simulink model "MixerSimple_LogIMU_RawDatas_30f4012"  (Simulink 7.2)
settings: Solver=FixedStepDiscrete  StartTime=0.0  StopTime=10.0  FixedStep=0.001  RelTol=1e-3
undefined symbols (not defined in the file or in its folder): IC1max, PWM
libraries: dsPICdrivers x42, simulink x31
CloseFcn:
  | rtwprivate ssgencode ModelCloseRequest Autopilote_30f4012
settings Model: Creator=Lubin  LastModifiedBy=Administrateur
settings OptimizationCC: InlineParams=on  InitFltsAndDblsToZero=on  OptimizeModelRefInitCode=on  LifeSpan=1
settings DebuggingCC: SaveWithParameterizedLinksMsg=none
settings HardwareCC: ProdBitPerInt=16  ProdEndianess=LittleEndian  ProdWordSize=16  ProdHWDeviceType=16-bit Generic
settings RTWCC: SystemTargetFile=dspic.tlc  TemplateMakefile=dspic_pic30_gcc.tmf  PostCodeGenCommand=dsPIC_Compile()  Description=Embedded Target for Microchip dsPIC (real-time)  GenerateReport=on  ProcessScript=dspic_make_rtw_hook  IncludeHyperlinkInReport=on  LaunchReport=on  GenerateTraceInfo=on  GenerateTraceReport=on  GenerateTraceReportSl=on  GenerateTraceReportSf=on  GenerateTraceReportEml=on
settings CodeAppCC: IgnoreCustomStorageClasses=off
settings STFCustomTargetCC: ModelReferenceCompliant=off  IncludeMdlTerminateFcn=off  CombineOutputUpdateFcns=on  SuppressErrorStatus=on  ERTCustomFileBanners=on  SupportContinuousTime=off  SupportNonInlinedSFcns=off  CPPClassGenCompliant=on  SystemTargetFile=dspic.tlc
settings ERTTargetCC: MultiwordLength=2048  ModelReferenceCompliant=off  CompOptLevelCompliant=off  IncludeMdlTerminateFcn=off  SuppressErrorStatus=on  ERTFirstTimeCompliant=off  ModelStepFunctionPrototypeControlCompliant=off  InlinedParameterPlacement=NonHierarchical  ERTSrcFileBannerTemplate=dsPIC_code_template.cgt  ERTHdrFileBannerTemplate=dsPIC_code_template.cgt  ERTDataSrcFileTemplate=dsPIC_code_template.cgt  ERTDataHdrFileTemplate=dsPIC_code_template.cgt  ERTCustomFileTemplate=dsPIC_main.tlc
settings CustomProperty: DataType=string  Value=C:\PROGRA~1\MATLAB\R2008a\bin\win32\gmake

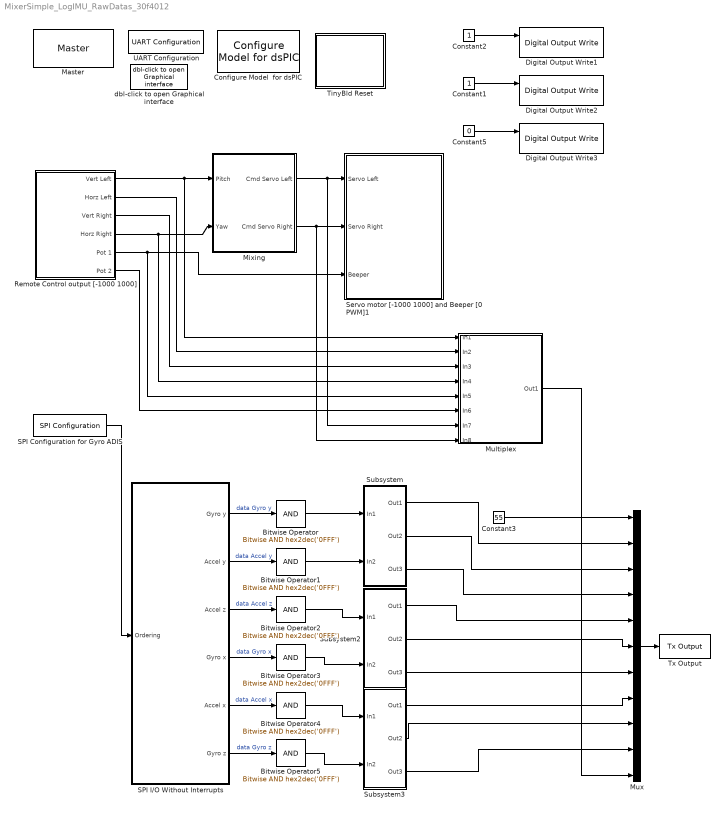
== system MixerSimple_LogIMU_RawDatas_30f4012 ==
  Bitwise Operator{,1..5} (6 alike) : simulink/Logic and Bit Operations/Bitwise Operator  logicop=AND  UseBitMask=on  BitMask=hex2dec('0FFF')  BitMaskRealWorld=Stored Integer
  Configure Model  for dsPIC : dsPICdrivers/Simulink Configuration/Configure Model  for dsPIC
  Constant1 : Constant  OutDataTypeMode=boolean  OutDataType=sfix(16)  OutScaling=2^0  OutDataTypeStr=boolean
  Constant2 : Constant  OutDataTypeMode=boolean  OutDataType=sfix(16)  OutScaling=2^0  OutDataTypeStr=boolean
  Constant3 : Constant  Value=55  OutDataTypeMode=uint8  OutDataType=sfix(16)  OutScaling=2^0  OutDataTypeStr=uint8  SampleTime=-1
  Constant5 : Constant  Value=0  OutDataTypeMode=boolean  OutDataType=sfix(16)  OutScaling=2^0  OutDataTypeStr=boolean
  Digital Output Write1 : dsPICdrivers/Digital I//O/Digital Output Write  Tag=dsPIC_Digital_Output  Priority=5  PORT=E  Pin=5  Simultaneous=off  OrderingInOutPopup=Input & Output
  Digital Output Write2 : dsPICdrivers/Digital I//O/Digital Output Write  Tag=dsPIC_Digital_Output  Priority=5  PORT=E  Pin=3  Simultaneous=off  OrderingInOutPopup=Input & Output
  Digital Output Write3 : dsPICdrivers/Digital I//O/Digital Output Write  Tag=dsPIC_Digital_Output  Priority=5  PORT=E  Pin=1  Simultaneous=off  OrderingInOutPopup=Input
  Master : dsPICdrivers/Master  Tag=dsPIC_MASTER  Priority=1  TimeStepType=Timer1  picType=30f4012  fcy=20e6  Quartz_33f=5e6  PLLActive_33f=off  fcyDesired_33f=0  tmr1="[1  19999  0]"  tmr1Info="Time Step : 0.001  ;   Error : 0%  PR1=19999"  tmr2345="[1  0  0  0]"  tmr2345cfg=[-1 -1 -1 -1]  IOautoConf=on  typePort="[ 0   0   0   0   0   0   0   0   0   0   0   0   0   0   0   0  10   0  13  13   6   6   0   0   0   0   0   0   0   0   0   0   0   0   0   0   0   0   0   0   0   0   0   0   0   5   4   0   6   6   0   0   0   0   0   0   0   0   0   0   0   0   0   0  11  10  11  10  11  10   0   0  17   0   0   0   0   0   0   0   0   0  14  15   0   0   0   0   0   0   0   0   0   0   0   0   0   0   0   0   0   0   0   0   0   0   0   0   0   0   0   0 ]"  TRIS="[ 65535  65534  65535  65535  65493  65535  65535 ]"  ADPCFG=61  MasterBusyPort=None  MasterOverloadPort=None  FOSC=XT_PLL8  ClockSwitchMonitor=Both disabled  TempProtection_33f=TEMP_ON  FPBOR=PBOR_OFF  PWRT=PWRT_4  MCLR=MCLR_DIS  PowerSave=off  OverrideFcy=off  NewFcy=1e6
  Mixing : Subsystem
  Multiplex : Subsystem
  Mux : Mux  Inputs=11
  Remote Control output [-1000 1000] : Subsystem
  SPI Configuration for Gyro ADIS : dsPICdrivers/SPI PORT/SPI Configuration  Tag=dsPIC_config_SPI  Priority=2  ConfigurationTime=At block execution (reconfigure on the fly)  OrderingInOutPopup=Output  SampleTime=-1  Frame_Enable=0  Frame_Sync=0  SPI=1  MODE=MASTER  USER_SCALER=2  StartEnable=Enable  SDO_EN=on  DATA_LENGTH=16 bits  SS_EN=off  SMP=Middle of bit  CKP=high  CKE=Idle to Active  Status="OK - Mode 1  -    Fsck= 10000000Hz"
  SPI I/O Without Interrupts : Subsystem
  Servo motor [-1000 1000] and Beeper [0 PWM]1 : Subsystem
  Subsystem : Subsystem
  Subsystem2 : Subsystem
  Subsystem3 : Subsystem
  TinyBld Reset : Subsystem  AncestorBlock=dsPICdrivers/OTHERS/TinyBld Reset
      mask Display: fprintf('TinyBld\nReset')
  Tx Output : dsPICdrivers/Serial PORT/Tx Output  Tag=dsPIC_TX  Priority=5  UART=1  OrderingInOutPopup=None
  UART Configuration : dsPICdrivers/Serial PORT/UART Configuration  Tag=dsPIC_config_UART  Priority=2  UART=1  proposed_BAUD=115200  ALT_TX_RX=on  InterruptTxWhen=When Transmit Buffer is empty  TXInterruptPri=1  TxBufferSize=32  TXEN=on  InterruptRxWhen=When Receive Buffer is full (contain 4 characters)  RXInterruptPri=1  RxBufferSize=32  BAUD=115200  UxBRG=10  Info="UxBRG = 10   ||  Real Baud : 113636   ||  % error : -1.3573  ||  max 11.3636 Bytes / Step"  RealBaud=0
  dbl-click to open Graphical interface : dsPICdrivers/Serial PORT/dbl-click to open Graphical interface  SystemSampleTime=-1  Nothing=0
  wires:
  Constant2/1 -> Digital Output Write1/1
  Constant1/1 -> Digital Output Write2/1
  Constant5/1 -> Digital Output Write3/1
  SPI Configuration for Gyro ADIS/1 -> SPI I/O Without Interrupts/1(Ordering)
  SPI I/O Without Interrupts/1(Gyro y) -> Bitwise Operator/1  "data Gyro y"
  SPI I/O Without Interrupts/2(Accel y) -> Bitwise Operator1/1  "data Accel y"
  SPI I/O Without Interrupts/3(Accel z) -> Bitwise Operator2/1  "data Accel z"
  SPI I/O Without Interrupts/4(Gyro x) -> Bitwise Operator3/1  "data Gyro x"
  SPI I/O Without Interrupts/5(Accel x) -> Bitwise Operator4/1  "data Accel x"
  SPI I/O Without Interrupts/6(Gyro z) -> Bitwise Operator5/1  "data Gyro z"
  Bitwise Operator/1 -> Subsystem/1(In1)
  Bitwise Operator1/1 -> Subsystem/2(In2)
  Bitwise Operator2/1 -> Subsystem2/1(In1)
  Bitwise Operator3/1 -> Subsystem2/2(In2)
  Bitwise Operator4/1 -> Subsystem3/1(In1)
  Bitwise Operator5/1 -> Subsystem3/2(In2)
  Mux/1 -> Tx Output/1
  Constant3/1 -> Mux/1
  Subsystem/1(Out1) -> Mux/2
  Subsystem/2(Out2) -> Mux/3
  Subsystem/3(Out3) -> Mux/4
  Subsystem2/1(Out1) -> Mux/5
  Subsystem2/2(Out2) -> Mux/6
  Subsystem2/3(Out3) -> Mux/7
  Subsystem3/1(Out1) -> Mux/8
  Subsystem3/2(Out2) -> Mux/9
  Subsystem3/3(Out3) -> Mux/10
  Mixing/1(Cmd Servo Left) -> Servo motor [-1000 1000] and Beeper [0 PWM]1/1(Servo Left), Multiplex/7(In7)
  Remote Control output [-1000 1000]/1(Vert Left) -> Mixing/1(Pitch), Multiplex/1(In1)
  Remote Control output [-1000 1000]/4(Horz Right) -> Mixing/2(Yaw), Multiplex/4(In4)
  Mixing/2(Cmd Servo Right) -> Servo motor [-1000 1000] and Beeper [0 PWM]1/2(Servo Right), Multiplex/8(In8)
  Remote Control output [-1000 1000]/5(Pot 1) -> Servo motor [-1000 1000] and Beeper [0 PWM]1/3(Beeper), Multiplex/5(In5)
  Remote Control output [-1000 1000]/2(Horz Left) -> Multiplex/2(In2)
  Remote Control output [-1000 1000]/3(Vert Right) -> Multiplex/3(In3)
  Remote Control output [-1000 1000]/6(Pot 2) -> Multiplex/6(In6)
  Multiplex/1(Out1) -> Mux/11

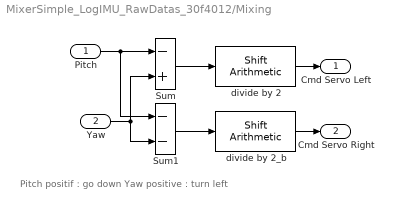
== system MixerSimple_LogIMU_RawDatas_30f4012/Mixing ==
  note: Pitch positif : go down
      | Yaw positive : turn left
  Pitch : Inport
  Yaw : Inport  Port=2
  Sum : Sum  Inputs=-+  AccumDataTypeStr=int16  OutDataTypeMode=int16  OutDataType=sfix(16)  OutScaling=2^0  OutDataTypeStr=int16  SaturateOnIntegerOverflow=on  InputSameDT=on
  Sum1 : Sum  Inputs=--  AccumDataTypeStr=int16  OutDataTypeMode=int16  OutDataType=sfix(16)  OutScaling=2^0  OutDataTypeStr=int16  SaturateOnIntegerOverflow=on  InputSameDT=on
  divide by 2 : simulink/Logic and Bit Operations/Shift Arithmetic  SystemSampleTime=-1  nBitShiftRight=1  nBinPtShiftRight=0
  divide by 2_b : simulink/Logic and Bit Operations/Shift Arithmetic  SystemSampleTime=-1  nBitShiftRight=1  nBinPtShiftRight=0
  Cmd Servo Left : Outport
  Cmd Servo Right : Outport  Port=2
  wires:
  divide by 2_b/1 -> Cmd Servo Right/1
  divide by 2/1 -> Cmd Servo Left/1
  Yaw/1 -> Sum/2, Sum1/2
  Sum1/1 -> divide by 2_b/1
  Sum/1 -> divide by 2/1
  Pitch/1 -> Sum/1, Sum1/1

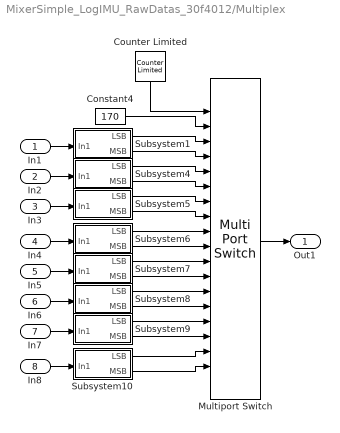
== system MixerSimple_LogIMU_RawDatas_30f4012/Multiplex ==
  In1 : Inport
  In2 : Inport  Port=2
  In3 : Inport  Port=3
  In4 : Inport  Port=4
  In5 : Inport  Port=5
  In6 : Inport  Port=6
  In7 : Inport  Port=7
  In8 : Inport  Port=8
  Constant4 : Constant  Value=170  OutDataTypeMode=uint8  OutDataType=sfix(16)  OutScaling=2^0  OutDataTypeStr=uint8  SampleTime=-1
  Counter Limited : simulink/Sources/Counter Limited  Orientation=down  SystemSampleTime=-1  uplimit=16  tsamp=-1
  Multiport Switch : MultiPortSwitch  Inputs=17  OutDataType=sfix(16)  OutScaling=2^0
  Subsystem1 : Subsystem
  Subsystem10 : Subsystem
  Subsystem4 : Subsystem
  Subsystem5 : Subsystem
  Subsystem6 : Subsystem
  Subsystem7 : Subsystem
  Subsystem8 : Subsystem
  Subsystem9 : Subsystem
  Out1 : Outport
  wires:
  Counter Limited/1 -> Multiport Switch/1
  Constant4/1 -> Multiport Switch/2
  Subsystem1/1(LSB) -> Multiport Switch/3
  Subsystem1/2(MSB) -> Multiport Switch/4
  Subsystem4/1(LSB) -> Multiport Switch/5
  Subsystem4/2(MSB) -> Multiport Switch/6
  Subsystem5/1(LSB) -> Multiport Switch/7
  Subsystem5/2(MSB) -> Multiport Switch/8
  Subsystem6/1(LSB) -> Multiport Switch/9
  Subsystem6/2(MSB) -> Multiport Switch/10
  Subsystem7/1(LSB) -> Multiport Switch/11
  Subsystem7/2(MSB) -> Multiport Switch/12
  Subsystem8/1(LSB) -> Multiport Switch/13
  Subsystem8/2(MSB) -> Multiport Switch/14
  Subsystem9/1(LSB) -> Multiport Switch/15
  Subsystem9/2(MSB) -> Multiport Switch/16
  Subsystem10/1(LSB) -> Multiport Switch/17
  Subsystem10/2(MSB) -> Multiport Switch/18
  In1/1 -> Subsystem1/1(In1)
  In2/1 -> Subsystem4/1(In1)
  In3/1 -> Subsystem5/1(In1)
  In4/1 -> Subsystem6/1(In1)
  Multiport Switch/1 -> Out1/1
  In5/1 -> Subsystem7/1(In1)
  In6/1 -> Subsystem8/1(In1)
  In7/1 -> Subsystem9/1(In1)
  In8/1 -> Subsystem10/1(In1)

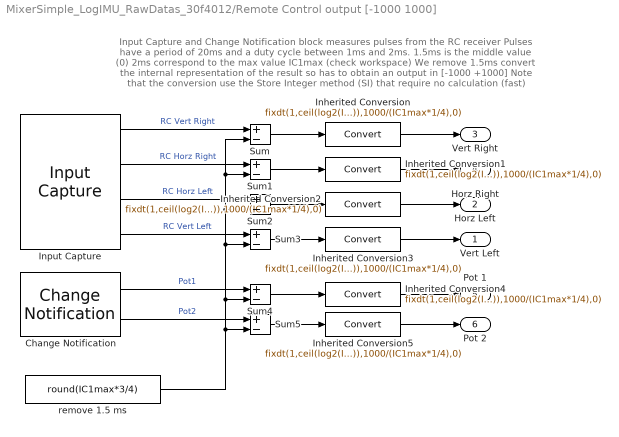
== system MixerSimple_LogIMU_RawDatas_30f4012/Remote Control output [-1000 1000] ==
  note: Input Capture and Change Notification block measures pulses from the RC receiver
      | Pulses have a period of 20ms and a duty cycle between 1ms and 2ms. 1.5ms is the middle value (0)
      | 2ms correspond to the max value IC1max (check workspace)
      | We remove 1.5ms convert the internal representation of the result so has to obtain an output in [-1000 +1000]
      | Note that the conversion use the Store Integer method (SI) that require no calculation (fast)
  Change Notification : dsPICdrivers/Peripheral I//O/Change Notification  Tag=dsPIC_PWM_CN  Priority=5  IntPriority=7  Channel="[4 5  ]"  Pin="[2  3]"  NumPort="[1  1]"  Channel_UP_Down_Periode="[1  1]"  MaxChannel="[0.002       0.002]"  SafeMarge="[10  10]"  MaxName=' CN4max , CN5max '  Precision="[15.2877      15.2877]"  Timer="[2  2]"  ChangeDetected="[0  0]"  PullUp="[0  0]"  SampleTime=.001  Status=OK
  Inherited Conversion{,1..5} (6 alike) : DataTypeConversion  OutDataTypeMode=Specify via dialog  OutDataType=fixdt(1,ceil(log2(IC1max*1/4)),1000/(IC1max*1/4),0)  OutDataTypeStr=fixdt(1,ceil(log2(IC1max*1/4)),1000/(IC1max*1/4),0)  ConvertRealWorld=Stored Integer (SI)  LockScale=on
  Input Capture : dsPICdrivers/Peripheral I//O/Input Capture  Tag=dsPIC_PWM_IC  Priority=5  IntPriority=7  Channel=[1 2 7 8 ]  Channel_UP_Down_Periode="[1  1  1  1]"  MaxChannel="[0.002       0.002       0.002       0.002]"  SafeMarge="[10  10  10  10]"  MaxName=' IC1max , IC2max , IC7max , IC8max '  Precision="[15.2877      15.2877      15.2877      15.2877]"  Timer="[2  2  2  2]"  ChangeDetected="[0  0  0  0]"  ChangeDetectedPortRef=0  SampleTime=.001  Status=OK
  Sum{,1..5} (6 alike) : Sum  Inputs=+-  AccumDataTypeStr=uint16  OutDataTypeMode=int16  OutDataType=sfix(16)  OutScaling=2^0  OutDataTypeStr=int16  InputSameDT=on
  remove 1.5 ms : Constant  Value=round(IC1max*3/4)  OutDataTypeMode=uint16  OutDataType=sfix(16)  OutScaling=2^0  OutDataTypeStr=uint16
  Vert Left : Outport
  Horz Left : Outport  Port=2
  Vert Right : Outport  Port=3
  Horz Right : Outport  Port=4
  Pot 1 : Outport  Port=5
  Pot 2 : Outport  Port=6
  wires:
  Input Capture/1 -> Sum/1  "RC Vert Right"
  Input Capture/2 -> Sum1/1  "RC Horz Right"
  Input Capture/3 -> Sum2/1  "RC Horz Left"
  Input Capture/4 -> Sum3/1  "RC Vert Left"
  Change Notification/1 -> Sum4/1  "Pot1"
  Change Notification/2 -> Sum5/1  "Pot2"
  remove 1.5 ms/1 -> Sum5/2, Sum/2, Sum1/2, Sum2/2, Sum3/2, Sum4/2
  Sum/1 -> Inherited Conversion/1
  Inherited Conversion/1 -> Vert Right/1
  Sum3/1 -> Inherited Conversion3/1
  Sum1/1 -> Inherited Conversion1/1
  Sum2/1 -> Inherited Conversion2/1
  Inherited Conversion1/1 -> Horz Right/1
  Inherited Conversion2/1 -> Horz Left/1
  Inherited Conversion3/1 -> Vert Left/1
  Sum4/1 -> Inherited Conversion4/1
  Sum5/1 -> Inherited Conversion5/1
  Inherited Conversion4/1 -> Pot 1/1
  Inherited Conversion5/1 -> Pot 2/1

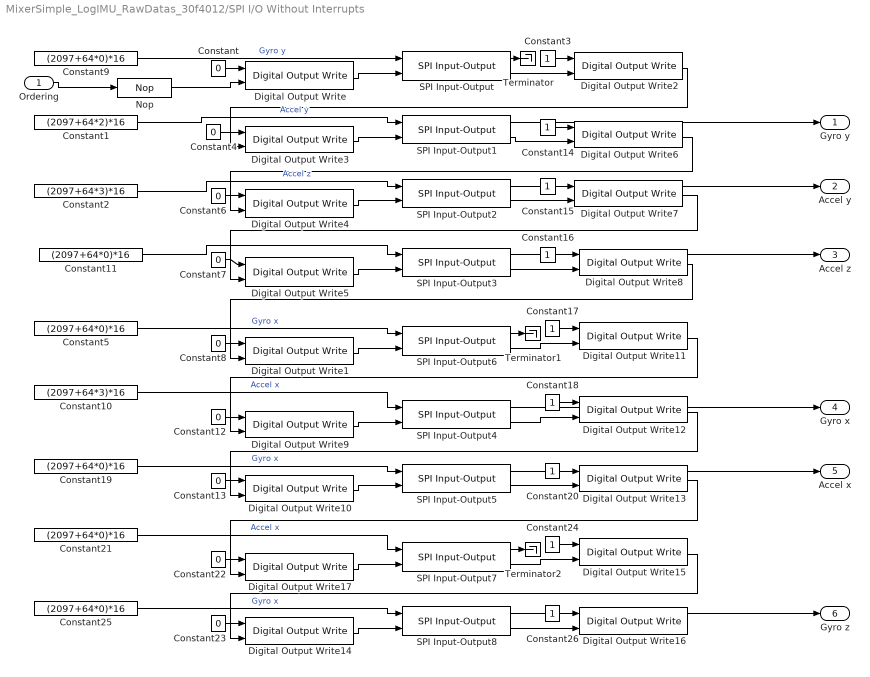
== system MixerSimple_LogIMU_RawDatas_30f4012/SPI I/O Without Interrupts ==
  Ordering : Inport  OutDataType=sfix(16)  OutScaling=2^0
  Constant{,4,6..8,12..13,22..23} (9 alike) : Constant  Value=0  OutDataTypeMode=boolean  OutDataType=sfix(16)  OutScaling=2^0  OutDataTypeStr=boolean
  Constant1 : Constant  Value=(2097+64*2)*16  VectorParams1D=off  OutDataTypeMode=uint16  OutDataType=sfix(16)  OutScaling=2^0  OutDataTypeStr=uint16  SampleTime=-1
  Constant10 : Constant  Value=(2097+64*3)*16  VectorParams1D=off  OutDataTypeMode=uint16  OutDataType=sfix(16)  OutScaling=2^0  OutDataTypeStr=uint16  SampleTime=-1
  Constant{5,9,11,19,21,25} (6 alike) : Constant  Value=(2097+64*0)*16  VectorParams1D=off  OutDataTypeMode=uint16  OutDataType=sfix(16)  OutScaling=2^0  OutDataTypeStr=uint16  SampleTime=-1
  Constant{3,14..18,20,24,26} (9 alike) : Constant  OutDataTypeMode=boolean  OutDataType=sfix(16)  OutScaling=2^0  OutDataTypeStr=boolean
  Constant2 : Constant  Value=(2097+64*3)*16  VectorParams1D=off  OutDataTypeMode=uint16  OutDataType=sfix(16)  OutScaling=2^0  OutDataTypeStr=uint16  SampleTime=-1
  Digital Output Write{,2..8} (8 alike) : dsPICdrivers/Digital I//O/Digital Output Write  Tag=dsPIC_Digital_Output  Priority=5  PORT=E  Pin=5  Simultaneous=off  OrderingInOutPopup=Input & Output
  Digital Output Write{1,9..13} (6 alike) : dsPICdrivers/Digital I//O/Digital Output Write  Tag=dsPIC_Digital_Output  Priority=5  PORT=E  Pin=3  Simultaneous=off  OrderingInOutPopup=Input & Output
  Digital Output Write14 : dsPICdrivers/Digital I//O/Digital Output Write  Tag=dsPIC_Digital_Output  Priority=5  PORT=B  Pin=0  Simultaneous=off  OrderingInOutPopup=Input & Output
  Digital Output Write15 : dsPICdrivers/Digital I//O/Digital Output Write  Tag=dsPIC_Digital_Output  Priority=5  PORT=B  Pin=0  Simultaneous=off  OrderingInOutPopup=Input & Output
  Digital Output Write16 : dsPICdrivers/Digital I//O/Digital Output Write  Tag=dsPIC_Digital_Output  Priority=5  PORT=B  Pin=0  Simultaneous=off  OrderingInOutPopup=Input
  Digital Output Write17 : dsPICdrivers/Digital I//O/Digital Output Write  Tag=dsPIC_Digital_Output  Priority=5  PORT=B  Pin=0  Simultaneous=off  OrderingInOutPopup=Input & Output
  Nop : dsPICdrivers/OTHERS/Nop  Tag=dsPIC_Reset  NbrNop=30
  SPI Input-Output{,1..8} (9 alike) : dsPICdrivers/SPI PORT/SPI Input-Output  Tag=dsPIC_SPI  SPI=1  INPUT=on  RESET_INPUT=off  OUTPUT=on  SPECIAL_SPI=Always Enable  DATA_LENGTH=16 bits  WAIT_INPUTDATA=on  OrderingInOutPopup=Input & Output  SampleTime=-1
  Terminator : Terminator
  Terminator1 : Terminator
  Terminator2 : Terminator
  Gyro y : Outport
  Accel y : Outport  Port=2
  Accel z : Outport  Port=3
  Gyro x : Outport  Port=4
  Accel x : Outport  Port=5
  Gyro z : Outport  Port=6
  wires:
  SPI Input-Output6/1 -> Terminator1/1
  SPI Input-Output/1 -> Terminator/1
  SPI Input-Output5/1 -> Accel x/1
  SPI Input-Output4/1 -> Gyro x/1
  SPI Input-Output3/1 -> Accel z/1
  SPI Input-Output2/1 -> Accel y/1
  SPI Input-Output1/1 -> Gyro y/1
  Digital Output Write12/1 -> Digital Output Write10/2
  Digital Output Write11/1 -> Digital Output Write9/2
  SPI Input-Output5/2 -> Digital Output Write13/2
  SPI Input-Output4/2 -> Digital Output Write12/2
  SPI Input-Output6/2 -> Digital Output Write11/2
  Constant20/1 -> Digital Output Write13/1
  Constant18/1 -> Digital Output Write12/1
  Constant17/1 -> Digital Output Write11/1
  Digital Output Write8/1 -> Digital Output Write1/2
  Digital Output Write10/1 -> SPI Input-Output5/2
  Digital Output Write9/1 -> SPI Input-Output4/2
  Digital Output Write1/1 -> SPI Input-Output6/2
  Constant13/1 -> Digital Output Write10/1
  Constant12/1 -> Digital Output Write9/1
  Constant8/1 -> Digital Output Write1/1
  Digital Output Write7/1 -> Digital Output Write5/2
  Digital Output Write6/1 -> Digital Output Write4/2
  SPI Input-Output3/2 -> Digital Output Write8/2
  SPI Input-Output2/2 -> Digital Output Write7/2
  Constant16/1 -> Digital Output Write8/1
  Constant15/1 -> Digital Output Write7/1
  SPI Input-Output1/2 -> Digital Output Write6/2
  Constant14/1 -> Digital Output Write6/1
  Digital Output Write2/1 -> Digital Output Write3/2
  Digital Output Write3/1 -> SPI Input-Output1/2
  Constant4/1 -> Digital Output Write3/1
  Digital Output Write5/1 -> SPI Input-Output3/2
  Constant7/1 -> Digital Output Write5/1
  Digital Output Write4/1 -> SPI Input-Output2/2
  Constant6/1 -> Digital Output Write4/1
  Digital Output Write/1 -> SPI Input-Output/2
  SPI Input-Output/2 -> Digital Output Write2/2
  Constant3/1 -> Digital Output Write2/1
  Constant/1 -> Digital Output Write/1
  Constant9/1 -> SPI Input-Output/1  "Gyro y"
  Constant1/1 -> SPI Input-Output1/1  "Accel y"
  Constant2/1 -> SPI Input-Output2/1  "Accel z"
  Constant11/1 -> SPI Input-Output3/1
  Constant5/1 -> SPI Input-Output6/1  "Gyro x"
  Constant10/1 -> SPI Input-Output4/1  "Accel x"
  Constant19/1 -> SPI Input-Output5/1  "Gyro x"
  Ordering/1 -> Nop/1
  Nop/1 -> Digital Output Write/2
  SPI Input-Output8/1 -> Gyro z/1
  Digital Output Write15/1 -> Digital Output Write14/2
  Digital Output Write13/1 -> Digital Output Write17/2
  SPI Input-Output8/2 -> Digital Output Write16/2
  SPI Input-Output7/2 -> Digital Output Write15/2
  Constant26/1 -> Digital Output Write16/1
  Constant24/1 -> Digital Output Write15/1
  Digital Output Write14/1 -> SPI Input-Output8/2
  Digital Output Write17/1 -> SPI Input-Output7/2
  Constant23/1 -> Digital Output Write14/1
  Constant22/1 -> Digital Output Write17/1
  Constant21/1 -> SPI Input-Output7/1  "Accel x"
  Constant25/1 -> SPI Input-Output8/1  "Gyro x"
  SPI Input-Output7/1 -> Terminator2/1

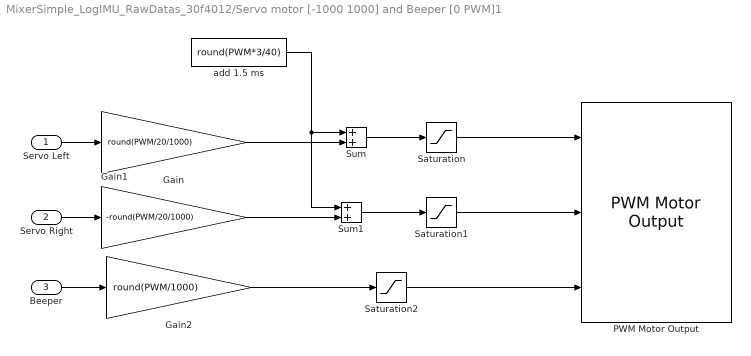
== system MixerSimple_LogIMU_RawDatas_30f4012/Servo motor [-1000 1000] and Beeper [0 PWM]1 ==
  Servo Left : Inport
  Servo Right : Inport  Port=2
  Beeper : Inport  Port=3
  Gain : Gain  Gain=round(PWM/20/1000)  ParameterDataType=sfix(16)  ParameterScaling=2^0  OutDataTypeMode=int16  OutDataType=sfix(16)  OutScaling=2^0  OutDataTypeStr=int16
  Gain1 : Gain  Gain=-round(PWM/20/1000)  ParameterDataType=sfix(16)  ParameterScaling=2^0  OutDataTypeMode=int16  OutDataType=sfix(16)  OutScaling=2^0  OutDataTypeStr=int16
  Gain2 : Gain  Gain=round(PWM/1000)  ParameterDataType=sfix(16)  ParameterScaling=2^0  OutDataTypeMode=uint16  OutDataType=sfix(16)  OutScaling=2^0  OutDataTypeStr=uint16  SaturateOnIntegerOverflow=on
  PWM Motor Output : dsPICdrivers/Peripheral I//O/PWM Motor Output  Tag=dsPIC_PWM_Motor  Priority=5  InputEnableChk=off  InputPeriodeChk=off  Channel=[1 2 3]  TPeriode=.02  PrescalerValue=16  PeriodeInteger=25000  MaxName='PWM'  Centered=off  HChannelON=off  Info="Nbr Bits : 15.6096  ||  PWM = 50000  ||  Prescaler = 16"  Delay=0  IntPriority=5  nbrPwmChannelPIC=3  Status=OK
  Saturation : Saturate  UpperLimit=2*PWM/20  LowerLimit=1*PWM/20  OutDataType=sfix(16)  OutScaling=2^0
  Saturation1 : Saturate  UpperLimit=2*PWM/20  LowerLimit=1*PWM/20  OutDataType=sfix(16)  OutScaling=2^0
  Saturation2 : Saturate  UpperLimit=PWM  LowerLimit=0  OutDataType=sfix(16)  OutScaling=2^0
  Sum : Sum  AccumDataTypeStr=int16  OutDataTypeMode=uint16  OutDataType=sfix(16)  OutScaling=2^0  OutDataTypeStr=uint16
  Sum1 : Sum  AccumDataTypeStr=int16  OutDataTypeMode=uint16  OutDataType=sfix(16)  OutScaling=2^0  OutDataTypeStr=uint16
  add 1.5 ms : Constant  Value=round(PWM*3/40)  OutDataTypeMode=uint16  OutDataType=sfix(16)  OutScaling=2^0  OutDataTypeStr=uint16
  wires:
  Saturation1/1 -> PWM Motor Output/2
  Saturation/1 -> PWM Motor Output/1
  Saturation2/1 -> PWM Motor Output/3
  Gain2/1 -> Saturation2/1
  Beeper/1 -> Gain2/1
  add 1.5 ms/1 -> Sum1/1, Sum/1
  Gain/1 -> Sum/2
  Gain1/1 -> Sum1/2
  Sum1/1 -> Saturation1/1
  Sum/1 -> Saturation/1
  Servo Right/1 -> Gain1/1
  Servo Left/1 -> Gain/1

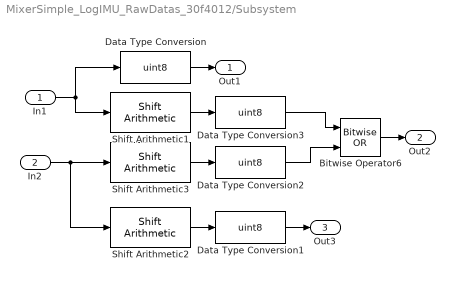
== system MixerSimple_LogIMU_RawDatas_30f4012/Subsystem ==
  In1 : Inport
  In2 : Inport  Port=2
  Bitwise Operator6 : simulink/Logic and Bit Operations/Bitwise Operator  logicop=OR  UseBitMask=off  NumInputPorts=2  BitMask=bin2dec('11011001')  BitMaskRealWorld=Stored Integer
  Data Type Conversion{,1..3} (4 alike) : DataTypeConversion  OutDataTypeMode=uint8  OutDataType=sfix(16)  OutScaling=2^0  OutDataTypeStr=uint8  ConvertRealWorld=Stored Integer (SI)
  Shift Arithmetic1 : simulink/Logic and Bit Operations/Shift Arithmetic  SystemSampleTime=-1  nBitShiftRight=8  nBinPtShiftRight=0
  Shift Arithmetic2 : simulink/Logic and Bit Operations/Shift Arithmetic  SystemSampleTime=-1  nBitShiftRight=4  nBinPtShiftRight=0
  Shift Arithmetic3 : simulink/Logic and Bit Operations/Shift Arithmetic  SystemSampleTime=-1  nBitShiftRight=-4  nBinPtShiftRight=0
  Out1 : Outport
  Out2 : Outport  Port=2
  Out3 : Outport  Port=3
  wires:
  Data Type Conversion3/1 -> Bitwise Operator6/1
  Data Type Conversion1/1 -> Out3/1
  Bitwise Operator6/1 -> Out2/1
  Data Type Conversion/1 -> Out1/1
  Shift Arithmetic1/1 -> Data Type Conversion3/1
  Data Type Conversion2/1 -> Bitwise Operator6/2
  Shift Arithmetic3/1 -> Data Type Conversion2/1
  Shift Arithmetic2/1 -> Data Type Conversion1/1
  In2/1 -> Shift Arithmetic2/1, Shift Arithmetic3/1
  In1/1 -> Data Type Conversion/1, Shift Arithmetic1/1

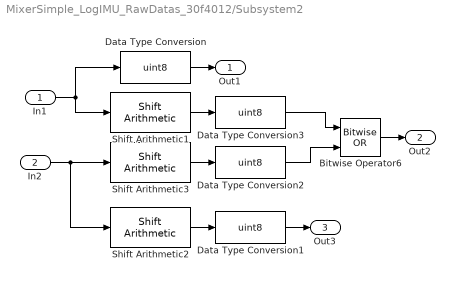
== system MixerSimple_LogIMU_RawDatas_30f4012/Subsystem2 ==
  In1 : Inport
  In2 : Inport  Port=2
  Bitwise Operator6 : simulink/Logic and Bit Operations/Bitwise Operator  logicop=OR  UseBitMask=off  NumInputPorts=2  BitMask=bin2dec('11011001')  BitMaskRealWorld=Stored Integer
  Data Type Conversion{,1..3} (4 alike) : DataTypeConversion  OutDataTypeMode=uint8  OutDataType=sfix(16)  OutScaling=2^0  OutDataTypeStr=uint8  ConvertRealWorld=Stored Integer (SI)
  Shift Arithmetic1 : simulink/Logic and Bit Operations/Shift Arithmetic  SystemSampleTime=-1  nBitShiftRight=8  nBinPtShiftRight=0
  Shift Arithmetic2 : simulink/Logic and Bit Operations/Shift Arithmetic  SystemSampleTime=-1  nBitShiftRight=4  nBinPtShiftRight=0
  Shift Arithmetic3 : simulink/Logic and Bit Operations/Shift Arithmetic  SystemSampleTime=-1  nBitShiftRight=-4  nBinPtShiftRight=0
  Out1 : Outport
  Out2 : Outport  Port=2
  Out3 : Outport  Port=3
  wires:
  In1/1 -> Shift Arithmetic1/1, Data Type Conversion/1
  In2/1 -> Shift Arithmetic3/1, Shift Arithmetic2/1
  Shift Arithmetic2/1 -> Data Type Conversion1/1
  Shift Arithmetic3/1 -> Data Type Conversion2/1
  Data Type Conversion2/1 -> Bitwise Operator6/2
  Shift Arithmetic1/1 -> Data Type Conversion3/1
  Data Type Conversion/1 -> Out1/1
  Bitwise Operator6/1 -> Out2/1
  Data Type Conversion1/1 -> Out3/1
  Data Type Conversion3/1 -> Bitwise Operator6/1

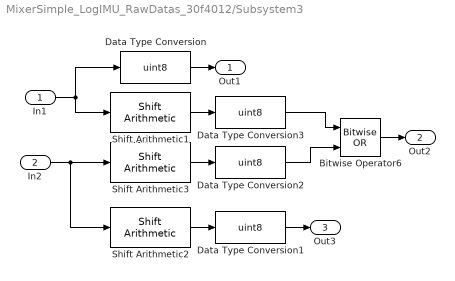
== system MixerSimple_LogIMU_RawDatas_30f4012/Subsystem3 ==
  In1 : Inport
  In2 : Inport  Port=2
  Bitwise Operator6 : simulink/Logic and Bit Operations/Bitwise Operator  logicop=OR  UseBitMask=off  NumInputPorts=2  BitMask=bin2dec('11011001')  BitMaskRealWorld=Stored Integer
  Data Type Conversion{,1..3} (4 alike) : DataTypeConversion  OutDataTypeMode=uint8  OutDataType=sfix(16)  OutScaling=2^0  OutDataTypeStr=uint8  ConvertRealWorld=Stored Integer (SI)
  Shift Arithmetic1 : simulink/Logic and Bit Operations/Shift Arithmetic  SystemSampleTime=-1  nBitShiftRight=8  nBinPtShiftRight=0
  Shift Arithmetic2 : simulink/Logic and Bit Operations/Shift Arithmetic  SystemSampleTime=-1  nBitShiftRight=4  nBinPtShiftRight=0
  Shift Arithmetic3 : simulink/Logic and Bit Operations/Shift Arithmetic  SystemSampleTime=-1  nBitShiftRight=-4  nBinPtShiftRight=0
  Out1 : Outport
  Out2 : Outport  Port=2
  Out3 : Outport  Port=3
  wires:
  Data Type Conversion3/1 -> Bitwise Operator6/1
  Data Type Conversion1/1 -> Out3/1
  Bitwise Operator6/1 -> Out2/1
  Data Type Conversion/1 -> Out1/1
  Shift Arithmetic1/1 -> Data Type Conversion3/1
  Data Type Conversion2/1 -> Bitwise Operator6/2
  Shift Arithmetic3/1 -> Data Type Conversion2/1
  Shift Arithmetic2/1 -> Data Type Conversion1/1
  In2/1 -> Shift Arithmetic2/1, Shift Arithmetic3/1
  In1/1 -> Data Type Conversion/1, Shift Arithmetic1/1

== system MixerSimple_LogIMU_RawDatas_30f4012/TinyBld Reset ==
  Compare To Constant : simulink/Logic and Bit Operations/Compare To Constant  SystemSampleTime=-1  relop===  const=55  LogicOutDataTypeMode=boolean  ZeroCross=off
  Enabled Subsystem : Subsystem  TreatAsAtomicUnit=on
  Logical Operator : Logic  AllPortsSameDT=off  OutDataTypeMode=boolean  OutDataTypeStr=boolean
  Logical Operator1 : Logic  Operator=OR  AllPortsSameDT=off  OutDataTypeMode=boolean  OutDataTypeStr=boolean
  Rx Input : dsPICdrivers/Serial PORT/Rx Input  Tag=dsPIC_RX  Priority=5  UART=1  SampleTime=.01  BlockingFctChk=off  OutputDefault=0  IsPresentFlagChk=on
  wires:
  Rx Input/1 -> Compare To Constant/1
  Compare To Constant/1 -> Logical Operator/1
  Rx Input/2 -> Logical Operator/2
  Logical Operator/1 -> Logical Operator1/1
  Logical Operator1/1 -> Enabled Subsystem/Enable

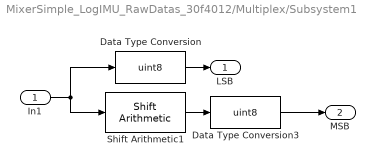
== system MixerSimple_LogIMU_RawDatas_30f4012/Multiplex/Subsystem1 ==
  In1 : Inport
  Data Type Conversion : DataTypeConversion  OutDataTypeMode=uint8  OutDataType=sfix(16)  OutScaling=2^0  OutDataTypeStr=uint8  ConvertRealWorld=Stored Integer (SI)
  Data Type Conversion3 : DataTypeConversion  OutDataTypeMode=uint8  OutDataType=sfix(16)  OutScaling=2^0  OutDataTypeStr=uint8  ConvertRealWorld=Stored Integer (SI)
  Shift Arithmetic1 : simulink/Logic and Bit Operations/Shift Arithmetic  SystemSampleTime=-1  nBitShiftRight=8  nBinPtShiftRight=0
  LSB : Outport
  MSB : Outport  Port=2
  wires:
  In1/1 -> Shift Arithmetic1/1, Data Type Conversion/1
  Shift Arithmetic1/1 -> Data Type Conversion3/1
  Data Type Conversion/1 -> LSB/1
  Data Type Conversion3/1 -> MSB/1

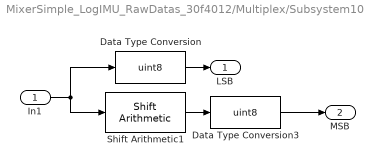
== system MixerSimple_LogIMU_RawDatas_30f4012/Multiplex/Subsystem10 ==
  In1 : Inport
  Data Type Conversion : DataTypeConversion  OutDataTypeMode=uint8  OutDataType=sfix(16)  OutScaling=2^0  OutDataTypeStr=uint8  ConvertRealWorld=Stored Integer (SI)
  Data Type Conversion3 : DataTypeConversion  OutDataTypeMode=uint8  OutDataType=sfix(16)  OutScaling=2^0  OutDataTypeStr=uint8  ConvertRealWorld=Stored Integer (SI)
  Shift Arithmetic1 : simulink/Logic and Bit Operations/Shift Arithmetic  SystemSampleTime=-1  nBitShiftRight=8  nBinPtShiftRight=0
  LSB : Outport
  MSB : Outport  Port=2
  wires:
  In1/1 -> Shift Arithmetic1/1, Data Type Conversion/1
  Shift Arithmetic1/1 -> Data Type Conversion3/1
  Data Type Conversion/1 -> LSB/1
  Data Type Conversion3/1 -> MSB/1

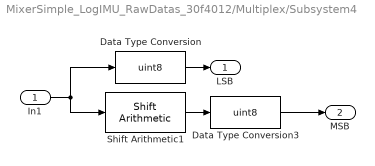
== system MixerSimple_LogIMU_RawDatas_30f4012/Multiplex/Subsystem4 ==
  In1 : Inport
  Data Type Conversion : DataTypeConversion  OutDataTypeMode=uint8  OutDataType=sfix(16)  OutScaling=2^0  OutDataTypeStr=uint8  ConvertRealWorld=Stored Integer (SI)
  Data Type Conversion3 : DataTypeConversion  OutDataTypeMode=uint8  OutDataType=sfix(16)  OutScaling=2^0  OutDataTypeStr=uint8  ConvertRealWorld=Stored Integer (SI)
  Shift Arithmetic1 : simulink/Logic and Bit Operations/Shift Arithmetic  SystemSampleTime=-1  nBitShiftRight=8  nBinPtShiftRight=0
  LSB : Outport
  MSB : Outport  Port=2
  wires:
  Data Type Conversion3/1 -> MSB/1
  Data Type Conversion/1 -> LSB/1
  Shift Arithmetic1/1 -> Data Type Conversion3/1
  In1/1 -> Data Type Conversion/1, Shift Arithmetic1/1

== system MixerSimple_LogIMU_RawDatas_30f4012/Multiplex/Subsystem5 ==
  In1 : Inport
  Data Type Conversion : DataTypeConversion  OutDataTypeMode=uint8  OutDataType=sfix(16)  OutScaling=2^0  OutDataTypeStr=uint8  ConvertRealWorld=Stored Integer (SI)
  Data Type Conversion3 : DataTypeConversion  OutDataTypeMode=uint8  OutDataType=sfix(16)  OutScaling=2^0  OutDataTypeStr=uint8  ConvertRealWorld=Stored Integer (SI)
  Shift Arithmetic1 : simulink/Logic and Bit Operations/Shift Arithmetic  SystemSampleTime=-1  nBitShiftRight=8  nBinPtShiftRight=0
  LSB : Outport
  MSB : Outport  Port=2
  wires:
  In1/1 -> Shift Arithmetic1/1, Data Type Conversion/1
  Shift Arithmetic1/1 -> Data Type Conversion3/1
  Data Type Conversion/1 -> LSB/1
  Data Type Conversion3/1 -> MSB/1

== system MixerSimple_LogIMU_RawDatas_30f4012/Multiplex/Subsystem6 ==
  In1 : Inport
  Data Type Conversion : DataTypeConversion  OutDataTypeMode=uint8  OutDataType=sfix(16)  OutScaling=2^0  OutDataTypeStr=uint8  ConvertRealWorld=Stored Integer (SI)
  Data Type Conversion3 : DataTypeConversion  OutDataTypeMode=uint8  OutDataType=sfix(16)  OutScaling=2^0  OutDataTypeStr=uint8  ConvertRealWorld=Stored Integer (SI)
  Shift Arithmetic1 : simulink/Logic and Bit Operations/Shift Arithmetic  SystemSampleTime=-1  nBitShiftRight=8  nBinPtShiftRight=0
  LSB : Outport
  MSB : Outport  Port=2
  wires:
  Data Type Conversion3/1 -> MSB/1
  Data Type Conversion/1 -> LSB/1
  Shift Arithmetic1/1 -> Data Type Conversion3/1
  In1/1 -> Data Type Conversion/1, Shift Arithmetic1/1

== system MixerSimple_LogIMU_RawDatas_30f4012/Multiplex/Subsystem7 ==
  In1 : Inport
  Data Type Conversion : DataTypeConversion  OutDataTypeMode=uint8  OutDataType=sfix(16)  OutScaling=2^0  OutDataTypeStr=uint8  ConvertRealWorld=Stored Integer (SI)
  Data Type Conversion3 : DataTypeConversion  OutDataTypeMode=uint8  OutDataType=sfix(16)  OutScaling=2^0  OutDataTypeStr=uint8  ConvertRealWorld=Stored Integer (SI)
  Shift Arithmetic1 : simulink/Logic and Bit Operations/Shift Arithmetic  SystemSampleTime=-1  nBitShiftRight=8  nBinPtShiftRight=0
  LSB : Outport
  MSB : Outport  Port=2
  wires:
  In1/1 -> Shift Arithmetic1/1, Data Type Conversion/1
  Shift Arithmetic1/1 -> Data Type Conversion3/1
  Data Type Conversion/1 -> LSB/1
  Data Type Conversion3/1 -> MSB/1

== system MixerSimple_LogIMU_RawDatas_30f4012/Multiplex/Subsystem8 ==
  In1 : Inport
  Data Type Conversion : DataTypeConversion  OutDataTypeMode=uint8  OutDataType=sfix(16)  OutScaling=2^0  OutDataTypeStr=uint8  ConvertRealWorld=Stored Integer (SI)
  Data Type Conversion3 : DataTypeConversion  OutDataTypeMode=uint8  OutDataType=sfix(16)  OutScaling=2^0  OutDataTypeStr=uint8  ConvertRealWorld=Stored Integer (SI)
  Shift Arithmetic1 : simulink/Logic and Bit Operations/Shift Arithmetic  SystemSampleTime=-1  nBitShiftRight=8  nBinPtShiftRight=0
  LSB : Outport
  MSB : Outport  Port=2
  wires:
  Data Type Conversion3/1 -> MSB/1
  Data Type Conversion/1 -> LSB/1
  Shift Arithmetic1/1 -> Data Type Conversion3/1
  In1/1 -> Data Type Conversion/1, Shift Arithmetic1/1

== system MixerSimple_LogIMU_RawDatas_30f4012/Multiplex/Subsystem9 ==
  In1 : Inport
  Data Type Conversion : DataTypeConversion  OutDataTypeMode=uint8  OutDataType=sfix(16)  OutScaling=2^0  OutDataTypeStr=uint8  ConvertRealWorld=Stored Integer (SI)
  Data Type Conversion3 : DataTypeConversion  OutDataTypeMode=uint8  OutDataType=sfix(16)  OutScaling=2^0  OutDataTypeStr=uint8  ConvertRealWorld=Stored Integer (SI)
  Shift Arithmetic1 : simulink/Logic and Bit Operations/Shift Arithmetic  SystemSampleTime=-1  nBitShiftRight=8  nBinPtShiftRight=0
  LSB : Outport
  MSB : Outport  Port=2
  wires:
  Data Type Conversion3/1 -> MSB/1
  Data Type Conversion/1 -> LSB/1
  Shift Arithmetic1/1 -> Data Type Conversion3/1
  In1/1 -> Data Type Conversion/1, Shift Arithmetic1/1

== system MixerSimple_LogIMU_RawDatas_30f4012/TinyBld Reset/Enabled Subsystem ==
  Enable : EnablePort
  While Iterator Subsystem : Subsystem  TreatAsAtomicUnit=on

== system MixerSimple_LogIMU_RawDatas_30f4012/TinyBld Reset/Enabled Subsystem/While Iterator Subsystem ==
  C1h : simulink/Logic and Bit Operations/Compare To Constant  SystemSampleTime=-1  relop===  const=66  LogicOutDataTypeMode=boolean  ZeroCross=off
  Logical Operator : Logic  Operator=NOT  AllPortsSameDT=off  OutDataTypeMode=boolean  OutDataTypeStr=boolean
  Rx Input : dsPICdrivers/Serial PORT/Rx Input  Tag=dsPIC_RX  Priority=5  UART=1  SampleTime=-1  BlockingFctChk=on  OutputDefault=0  IsPresentFlagChk=off
  Software RESET : S-Function  Tag=dsPIC_Reset  FunctionName=dsPIC_Reset  EnableBusSupport=off
      mask Description: Reset the microcontroller when input is different from 0
      mask Display:
      | fprintf('Reset');
      | port_label('input', 1 ,'~=0');
  While Iterator : WhileIterator  MaxIters=-1  WhileBlockType=do-while  ResetStates=reset
  wires:
  Logical Operator/1 -> While Iterator/1
  Rx Input/1 -> C1h/1
  C1h/1 -> Software RESET/1, Logical Operator/1
